simulink model "energy_trading"  (R2024b)
settings: Solver=VariableStepAuto  StartTime=0.0  StopTime=0.1  RelTol=1e-3
undefined symbols (not defined in the file): Acid, Lead
libraries: spsSeriesRLCBranchLib x12, spsPVArrayLib x3, spsDiodeLib x3, spsVoltageMeasurementLib x3, spsBatteryLib x2, spsMosfetLib x2, simulink x2, spsCurrentMeasurementLib x1, spsIGBTDiodeLib x1, spsPWMGenerator2LevelLib x1, spsUniversalBridgeLib x1, sps_lib x1
settings Model: Creator=ASUS  LastModifiedBy=ASUS

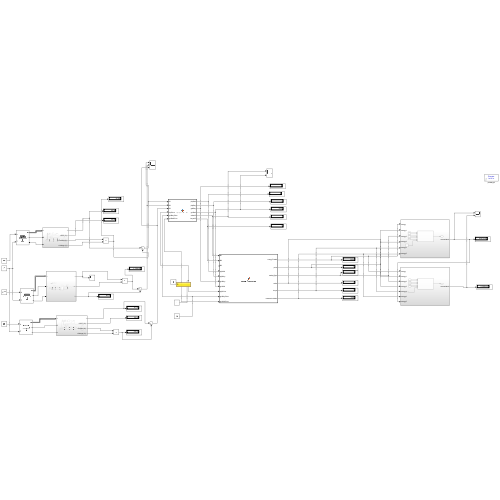
[thumbnail: Simulink's stored preview of the top-level diagram]
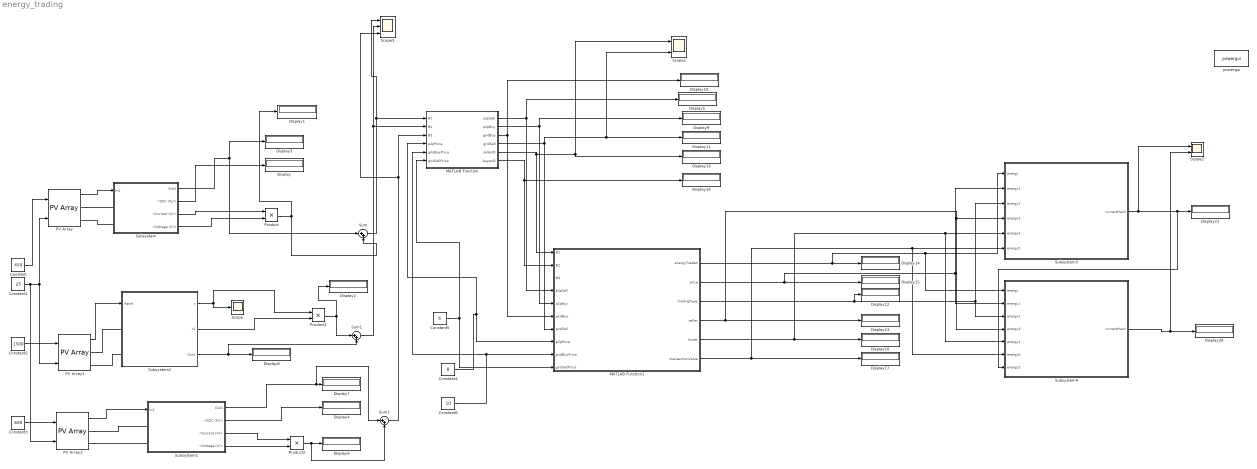
== system energy_trading ==
  Constant : Constant  Value=450
  Constant1 : Constant  Value=25
  Constant2 : Constant  Value=1500
  Constant3 : Constant  Value=600
  Constant4 : Constant  Value=8
  Constant5 : Constant  Value=6
  Constant6 : Constant  Value=10
  Display{,1..21} (22 alike) : Display
  MATLAB Function : MATLAB Function  TreatAsAtomicUnit=on
  MATLAB Function1 : MATLAB Function  TreatAsAtomicUnit=on
  PV Array : spsPVArrayLib/PV Array  Npar=1  Nser=1  PlotType=array @ 1000 W/m2 & specified temperatures  S_vec="[ 1000  500  100 ]"  Temp_C_vec="[ 45 25  ]"  ModuleName=User-defined  PlotWhenSelected=off  Pm=213.15  Ncell=60  Voc=36.3  Isc=7.84  Vm=29  Im=7.35  beta_Voc_pc=-0.36099  alpha_Isc_pc=0.102  beta_Voc=-0.13104  alpha_Isc=0.0079968  IL=7.8654  I0=2.9273e-10  nI=0.98119  Rsh=313.0553  Rs=0.39381  RobustModel=off  RobustCellTemperature=313.3991  BAL=on  Tc=1e-6  Tfilter=5e-5
  PV Array1 : spsPVArrayLib/PV Array  Npar=1  Nser=1  PlotType=array @ 1000 W/m2 & specified temperatures  S_vec="[ 1000  500  100 ]"  Temp_C_vec="[ 45 25  ]"  ModuleName=User-defined  PlotWhenSelected=off  Pm=213.15  Ncell=60  Voc=36.3  Isc=7.84  Vm=29  Im=7.35  beta_Voc_pc=-0.36099  alpha_Isc_pc=0.102  beta_Voc=-0.13104  alpha_Isc=0.0079968  IL=7.8654  I0=2.9273e-10  nI=0.98119  Rsh=313.0553  Rs=0.39381  RobustModel=off  RobustCellTemperature=313.3991  BAL=on  Tc=1e-6  Tfilter=5e-5
  PV Array2 : spsPVArrayLib/PV Array  Npar=1  Nser=1  PlotType=array @ 1000 W/m2 & specified temperatures  S_vec="[ 1000  500  100 ]"  Temp_C_vec="[ 45 25  ]"  ModuleName=User-defined  PlotWhenSelected=off  Pm=213.15  Ncell=60  Voc=36.3  Isc=7.84  Vm=29  Im=7.35  beta_Voc_pc=-0.36099  alpha_Isc_pc=0.102  beta_Voc=-0.13104  alpha_Isc=0.0079968  IL=7.8654  I0=2.9273e-10  nI=0.98119  Rsh=313.0553  Rs=0.39381  RobustModel=off  RobustCellTemperature=313.3991  BAL=on  Tc=1e-6  Tfilter=5e-5
  Product : Product
  Product1 : Product
  Product2 : Product
  Scope : Scope
  Scope1 : Scope  NumInputPorts=2
  Scope2 : Scope  NumInputPorts=2
  Scope3 : Scope  NumInputPorts=3
  Subsystem : Subsystem
  Subsystem1 : Subsystem
  Subsystem2 : Subsystem
  Subsystem3 : Subsystem
  Subsystem4 : Subsystem
  Sum : Sum  Inputs=|++
  Sum1 : Sum  Inputs=|++
  Sum2 : Sum  Inputs=|++
  powergui : sps_lib/powergui  Priority=1  SimulationMode=Discrete  SampleTime=1e-06  frequency=60  Iterations=50  frequencyindice=0  Pbase=100e6  ErrMax=1e-4  UnitsV=kV  UnitsW=MW  buscounter=0  FunctionMessages=off  echomessages=off  EnableUseOfTLC=off  CurrentSourceSwitches=off  DisableSnubberDevices=off  DisableRonSwitches=off  DisableVfSwitches=off  DisplayEquations=off  AutomaticDiscreteSolvers=off  SolverType=Tustin/Backward Euler (TBE)  Interpol=off  ExternalGateDelay=off  methode=off  Ts=100  x0status=blocks  SPID=on  SwTol=0  HookPort=off  NonlinearTolerance=1e-4  nMaxIteration=100  ContinueOnMaxIteration=off  RestoreLinks=warning  ResistiveCurrentMeasurement=off  Frange=[0:2:500]  Ylog=off  Xlog=on  ShowGrid=off  save=off  variable=ZData  structure=0  ZoomFFT=off  StartTime=0.0  cycles=1  DisplayStyle=1  fundamental=60  FreqAxis=off  MaxFrequency=1000  frequencyindicesteady=1  RmsSteady=1  display=off
  wires:
  Constant/1 -> PV Array/1
  Constant1/1 -> PV Array2/2, PV Array1/2, PV Array/2
  Constant3/1 -> PV Array2/1
  Constant2/1 -> PV Array1/1
  PV Array/1 -> Subsystem/1(In1)
  Subsystem/1(Out1) -> Display3/1, Sum/1
  Subsystem/2(<SOC (%)>) -> Display/1
  Subsystem/3(<Current (A)>) -> Product/1
  Subsystem/4(<Voltage (V)>) -> Product/2
  PV Array2/1 -> Subsystem1/1(In1)
  Subsystem1/1(Out1) -> Sum2/1, Display7/1
  Subsystem1/2(<SOC (%)>) -> Display4/1
  Subsystem2/1(v) -> Scope/1, Product1/1
  Product/1 -> Sum/2, Display1/1
  Subsystem2/2(c1) -> Product1/2
  Product1/1 -> Sum1/1, Display2/1
  PV Array1/1 -> Subsystem2/1(Inport)
  Subsystem2/3(Out1) -> Sum1/2, Display8/1
  Product2/1 -> Sum2/2, Display6/1
  Subsystem1/3(<Current (A)>) -> Product2/1
  Subsystem1/4(<Voltage (V)>) -> Product2/2
  MATLAB Function/1(p2pSell) -> Display5/1, MATLAB Function1/4(p2pSell)
  MATLAB Function/2(p2pBuy) -> Display9/1, MATLAB Function1/5(p2pBuy)
  MATLAB Function/3(gridBuy) -> Display10/1, MATLAB Function1/6(gridBuy)
  MATLAB Function/4(gridSell) -> Scope1/2, Display11/1, MATLAB Function1/7(gridSell)
  Constant5/1 -> MATLAB Function/6(gridSellPrice), MATLAB Function1/10(gridSellPrice)
  Constant6/1 -> MATLAB Function/5(gridBuyPrice), MATLAB Function1/9(gridBuyPrice)
  Constant4/1 -> MATLAB Function/4(p2pPrice), MATLAB Function1/8(p2pPrice)
  MATLAB Function1/3(tradingType) -> Display12/1, Subsystem4/3(energy2), Subsystem3/3(energy2)
  MATLAB Function1/4(seller) -> Subsystem4/4(energy3), Subsystem3/4(energy3), Display13/1
  MATLAB Function1/1(energyTraded) -> Subsystem4/1(energy), Subsystem3/1(energy), Display14/1
  MATLAB Function1/2(price) -> Subsystem4/2(energy1), Subsystem3/2(energy1), Display15/1
  MATLAB Function1/5(buyer) -> Subsystem4/5(energy4), Subsystem3/5(energy4), Display16/1
  MATLAB Function1/6(transactionValue) -> Subsystem4/6(energy6), Subsystem3/6(energy5), Display17/1
  MATLAB Function/5(sellerID) -> MATLAB Function1/1(B1), Display19/1, Scope1/1
  MATLAB Function/6(buyerID) -> MATLAB Function1/2(B2), Display18/1
  Subsystem3/1(currentHash) -> Scope2/1, Subsystem4/7(energy5), Display21/1
  Subsystem4/1(currentHash) -> Scope2/2, Display20/1
  Sum/1 -> Scope3/1, MATLAB Function/1(B1)
  Sum1/1 -> Scope3/2, MATLAB Function/2(B2)
  Sum2/1 -> Scope3/3, MATLAB Function/3(B3)
  connections:
  PV Array/RConn1 -- Subsystem/LConn1
  Subsystem/LConn2 -- PV Array/RConn2
  PV Array2/RConn1 -- Subsystem1/LConn1
  PV Array2/RConn2 -- Subsystem1/LConn2
  PV Array1/RConn1 -- Subsystem2/LConn1
  Subsystem2/LConn2 -- PV Array1/RConn2

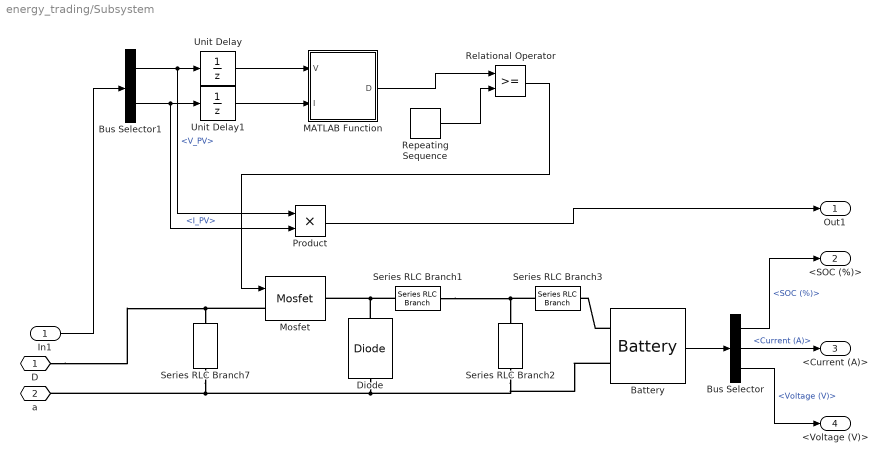
== system energy_trading/Subsystem ==
  In1 : Inport
  Battery : spsBatteryLib/Battery  BatType=Lead-Acid  NomV=12  NomQ=100  SOC=45  Batt_Tr=1  PresetModel=on  MaxQ=104.1667  MinV=9  FullV=13.0658  Dis_rate=20  R=0.0012  Normal_OP=31.0278  expZone="[12.2171     0.333333]"
  Bus Selector : BusSelector  OutputSignals=SOC (%),Current (A),Voltage (V)
  Bus Selector1 : BusSelector  OutputSignals=V_PV,I_PV
  Diode : spsDiodeLib/Diode  Ron=0.001  Lon=0  Vf=0.8  IC=0  UseSnubber=0  Rs=500  Cs=250e-9  Measurements=off
  MATLAB Function : MATLAB Function  TreatAsAtomicUnit=on
  Mosfet : spsMosfetLib/Mosfet  Ron=0.1  Lon=0  Rd=0.01  Vfd=0  IC=0  Rs=1e5  Cs=inf  Measurements=off
  Product : Product
  Relational Operator : RelationalOperator  OutDataTypeStr=boolean  RndMeth=Simplest  InputSameDT=off
  Repeating Sequence : simulink/Sources/Repeating Sequence  rep_seq_t=[0 0.0002]  rep_seq_y=[0 1]
  Series RLC Branch1 : spsSeriesRLCBranchLib/Series RLC Branch  LConnTagsString=__new0  RConnTagsString=__new0  BranchType=L  Resistance=0.0001  Inductance=0.783e-3  SetiL0=off  InitialCurrent=0  Capacitance=1000e-4  Setx0=off  InitialVoltage=0  Measurements=None
  Series RLC Branch2 : spsSeriesRLCBranchLib/Series RLC Branch  LConnTagsString=__new0  RConnTagsString=__new0  BranchType=C  Resistance=0.0001  Inductance=0.783e-3  SetiL0=off  InitialCurrent=0  Capacitance=364e-3  Setx0=off  InitialVoltage=0  Measurements=None
  Series RLC Branch3 : spsSeriesRLCBranchLib/Series RLC Branch  LConnTagsString=__new0  RConnTagsString=__new0  BranchType=R  Resistance=0.01  Inductance=0.783e-3  SetiL0=off  InitialCurrent=0  Capacitance=1000e-4  Setx0=off  InitialVoltage=0  Measurements=None
  Series RLC Branch7 : spsSeriesRLCBranchLib/Series RLC Branch  LConnTagsString=__new0  RConnTagsString=__new0  BranchType=RC  Resistance=0.0001  Inductance=1e-3  SetiL0=off  InitialCurrent=0  Capacitance=1000e-4  Setx0=off  InitialVoltage=0  Measurements=None
  Unit Delay : UnitDelay  SampleTime=1e-4  HasFrameUpgradeWarning=on
  Unit Delay1 : UnitDelay  SampleTime=1e-4  HasFrameUpgradeWarning=on
  D : PMIOPort  Side=Left
  a : PMIOPort  Port=2  Side=Left
  Out1 : Outport
  <SOC (%)> : Outport  Port=2
  <Current (A)> : Outport  Port=3
  <Voltage (V)> : Outport  Port=4
  wires:
  Battery/1 -> Bus Selector/1
  MATLAB Function/1(D) -> Relational Operator/1
  Bus Selector1/2 -> Product/2, Unit Delay1/1  "<I_PV>"
  Unit Delay1/1 -> MATLAB Function/2(I)
  Bus Selector1/1 -> Product/1, Unit Delay/1  "<V_PV>"
  Product/1 -> Out1/1
  Relational Operator/1 -> Mosfet/1
  Unit Delay/1 -> MATLAB Function/1(V)
  Repeating Sequence/1 -> Relational Operator/2
  Bus Selector/1 -> <SOC (%)>/1  "<SOC (%)>"
  In1/1 -> Bus Selector1/1
  Bus Selector/2 -> <Current (A)>/1  "<Current (A)>"
  Bus Selector/3 -> <Voltage (V)>/1  "<Voltage (V)>"
  connections:
  Series RLC Branch7/RConn1 -- a/RConn1 -- Battery/LConn2 -- Series RLC Branch2/LConn1 -- Diode/LConn1
  Series RLC Branch1/LConn1 -- Series RLC Branch2/RConn1 -- Series RLC Branch3/RConn1
  Diode/RConn1 -- Series RLC Branch1/RConn1 -- Mosfet/RConn1
  Battery/LConn1 -- Series RLC Branch3/LConn1
  Mosfet/LConn1 -- D/RConn1 -- Series RLC Branch7/LConn1

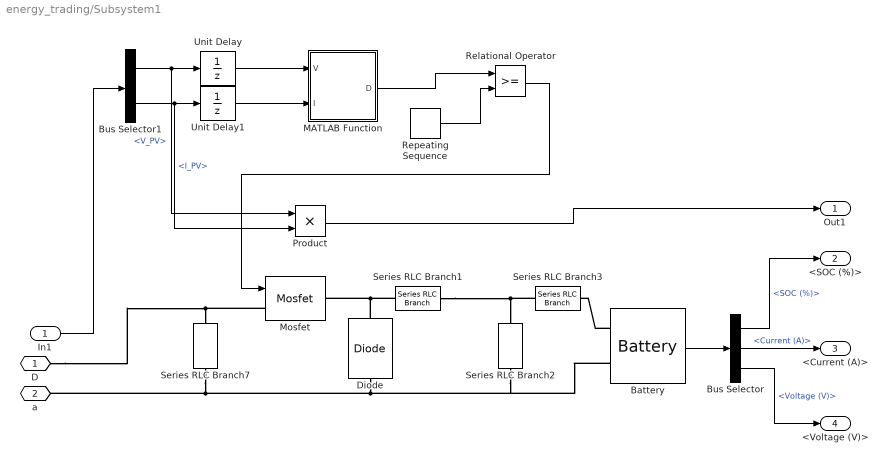
== system energy_trading/Subsystem1 ==
  In1 : Inport
  Battery : spsBatteryLib/Battery  BatType=Lead-Acid  NomV=12  NomQ=100  SOC=45  Batt_Tr=1  PresetModel=on  MaxQ=104.1667  MinV=9  FullV=13.0658  Dis_rate=20  R=0.0012  Normal_OP=31.0278  expZone="[12.2171     0.333333]"
  Bus Selector : BusSelector  OutputSignals=SOC (%),Current (A),Voltage (V)
  Bus Selector1 : BusSelector  OutputSignals=V_PV,I_PV
  Diode : spsDiodeLib/Diode  Ron=0.001  Lon=0  Vf=0.8  IC=0  UseSnubber=0  Rs=500  Cs=250e-9  Measurements=off
  MATLAB Function : MATLAB Function  TreatAsAtomicUnit=on
  Mosfet : spsMosfetLib/Mosfet  Ron=0.1  Lon=0  Rd=0.01  Vfd=0  IC=0  Rs=1e5  Cs=inf  Measurements=off
  Product : Product
  Relational Operator : RelationalOperator  OutDataTypeStr=boolean  RndMeth=Simplest  InputSameDT=off
  Repeating Sequence : simulink/Sources/Repeating Sequence  rep_seq_t=[0 0.0002]  rep_seq_y=[0 1]
  Series RLC Branch1 : spsSeriesRLCBranchLib/Series RLC Branch  LConnTagsString=__new0  RConnTagsString=__new0  BranchType=L  Resistance=0.0001  Inductance=0.783e-3  SetiL0=off  InitialCurrent=0  Capacitance=1000e-4  Setx0=off  InitialVoltage=0  Measurements=None
  Series RLC Branch2 : spsSeriesRLCBranchLib/Series RLC Branch  LConnTagsString=__new0  RConnTagsString=__new0  BranchType=C  Resistance=0.0001  Inductance=0.783e-3  SetiL0=off  InitialCurrent=0  Capacitance=364e-3  Setx0=off  InitialVoltage=0  Measurements=None
  Series RLC Branch3 : spsSeriesRLCBranchLib/Series RLC Branch  LConnTagsString=__new0  RConnTagsString=__new0  BranchType=R  Resistance=0.01  Inductance=0.783e-3  SetiL0=off  InitialCurrent=0  Capacitance=1000e-4  Setx0=off  InitialVoltage=0  Measurements=None
  Series RLC Branch7 : spsSeriesRLCBranchLib/Series RLC Branch  LConnTagsString=__new0  RConnTagsString=__new0  BranchType=RC  Resistance=0.0001  Inductance=1e-3  SetiL0=off  InitialCurrent=0  Capacitance=1000e-4  Setx0=off  InitialVoltage=0  Measurements=None
  Unit Delay : UnitDelay  SampleTime=1e-4  HasFrameUpgradeWarning=on
  Unit Delay1 : UnitDelay  SampleTime=1e-4  HasFrameUpgradeWarning=on
  D : PMIOPort  Side=Left
  a : PMIOPort  Port=2  Side=Left
  Out1 : Outport
  <SOC (%)> : Outport  Port=2
  <Current (A)> : Outport  Port=3
  <Voltage (V)> : Outport  Port=4
  wires:
  Battery/1 -> Bus Selector/1
  MATLAB Function/1(D) -> Relational Operator/1
  Bus Selector1/2 -> Product/2, Unit Delay1/1  "<I_PV>"
  Unit Delay1/1 -> MATLAB Function/2(I)
  Bus Selector1/1 -> Product/1, Unit Delay/1  "<V_PV>"
  Product/1 -> Out1/1
  Relational Operator/1 -> Mosfet/1
  Unit Delay/1 -> MATLAB Function/1(V)
  Repeating Sequence/1 -> Relational Operator/2
  Bus Selector/1 -> <SOC (%)>/1  "<SOC (%)>"
  In1/1 -> Bus Selector1/1
  Bus Selector/2 -> <Current (A)>/1  "<Current (A)>"
  Bus Selector/3 -> <Voltage (V)>/1  "<Voltage (V)>"
  connections:
  Series RLC Branch7/RConn1 -- Series RLC Branch2/LConn1 -- Battery/LConn2 -- Diode/LConn1 -- a/RConn1
  Series RLC Branch1/LConn1 -- Series RLC Branch3/RConn1 -- Series RLC Branch2/RConn1
  Diode/RConn1 -- Mosfet/RConn1 -- Series RLC Branch1/RConn1
  Battery/LConn1 -- Series RLC Branch3/LConn1
  Mosfet/LConn1 -- D/RConn1 -- Series RLC Branch7/LConn1

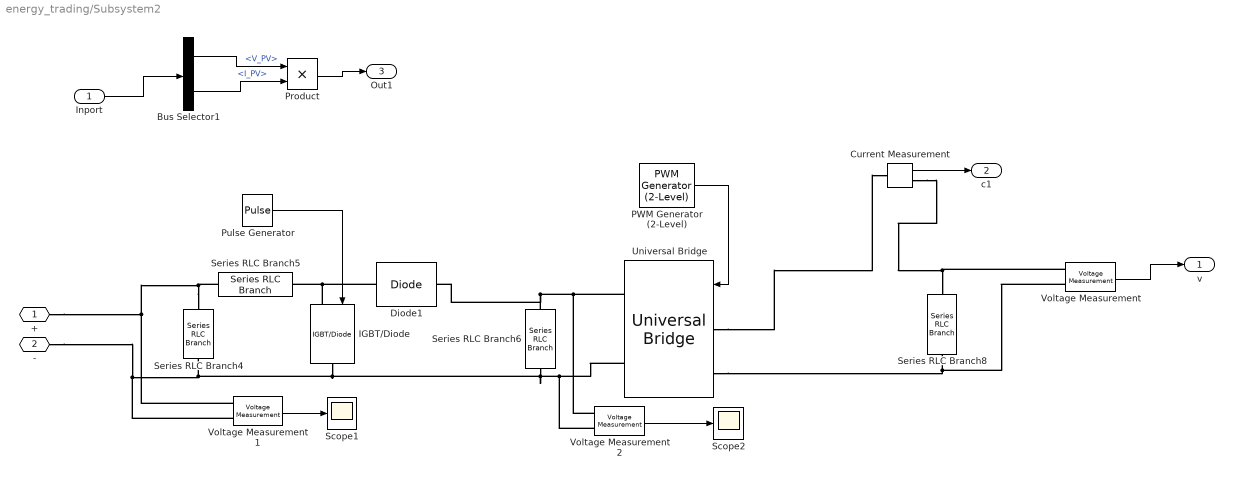
== system energy_trading/Subsystem2 ==
  Inport : Inport
  Bus Selector1 : BusSelector  OutputSignals=V_PV,I_PV
  Current Measurement : spsCurrentMeasurementLib/Current Measurement  PhasorSimulation=off  OutputType=Complex  PSBequivalent=0
  Diode1 : spsDiodeLib/Diode  Ron=0.001  Lon=0  Vf=0.8  IC=0  UseSnubber=0  Rs=500  Cs=250e-9  Measurements=off
  IGBT/Diode : spsIGBTDiodeLib/IGBT//Diode  Ron=1e-3  Rs=1e5  Cs=inf  Measurements=off
  PWM Generator (2-Level) : spsPWMGenerator2LevelLib/PWM Generator (2-Level)  ModulatorType=Single-phase full-bridge (4 pulses)  ModulatorMode=Unsynchronized  Fc=27*60  Pc=90  nF=27  MinMax="[ -1  1 ]"  SamplingTechnique=Natural  ModulatingSignals=on  m=0.8  Freq=60  Phase=0  Ts=0  ShowCarrierOutport=off
  Product : Product
  Pulse Generator : DiscretePulseGenerator  PulseType=Time based  Period=1/1500  PulseWidth=50
  Scope1 : Scope
  Scope2 : Scope
  Series RLC Branch4 : spsSeriesRLCBranchLib/Series RLC Branch  LConnTagsString=__new0  RConnTagsString=__new0  BranchType=C  Resistance=0.0001  Inductance=1e-3  SetiL0=off  InitialCurrent=0  Capacitance=0.006  Setx0=off  InitialVoltage=0  Measurements=None
  Series RLC Branch5 : spsSeriesRLCBranchLib/Series RLC Branch  LConnTagsString=__new0  RConnTagsString=__new0  BranchType=L  Resistance=0.0001  Inductance=0.02  SetiL0=off  InitialCurrent=0  Capacitance=0.006  Setx0=off  InitialVoltage=0  Measurements=None
  Series RLC Branch6 : spsSeriesRLCBranchLib/Series RLC Branch  LConnTagsString=__new0  RConnTagsString=__new0  BranchType=C  Resistance=0.0001  Inductance=1e-3  SetiL0=off  InitialCurrent=0  Capacitance=0.006  Setx0=off  InitialVoltage=0  Measurements=None
  Series RLC Branch8 : spsSeriesRLCBranchLib/Series RLC Branch  LConnTagsString=__new0  RConnTagsString=__new0  BranchType=L  Resistance=0.0001  Inductance=50  SetiL0=off  InitialCurrent=0  Capacitance=0.006  Setx0=off  InitialVoltage=0  Measurements=None
  Universal Bridge : spsUniversalBridgeLib/Universal Bridge  Arms=2  SnubberResistance=1e5  SnubberCapacitance=inf  Device=IGBT / Diodes  Ron=1e-3  Lon=0  ForwardVoltages="[  0  0  ]"  ForwardVoltage=0  GTOparameters=[ 10e-6 , 20e-6 ]  IGBTparameters=[ 1e-6 , 2e-6 ]  Measurements=None  Measurements_2=None  converterType=Rectifier
  Voltage Measurement : spsVoltageMeasurementLib/Voltage Measurement  PhasorSimulation=off  OutputType=Complex  PSBequivalent=0
  Voltage Measurement1 : spsVoltageMeasurementLib/Voltage Measurement  PhasorSimulation=off  OutputType=Complex  PSBequivalent=0
  Voltage Measurement2 : spsVoltageMeasurementLib/Voltage Measurement  PhasorSimulation=off  OutputType=Complex  PSBequivalent=0
  + : PMIOPort  Side=Left
  - : PMIOPort  Port=2  Side=Left
  v : Outport
  c1 : Outport  Port=2
  Out1 : Outport  Port=3
  wires:
  PWM Generator (2-Level)/1 -> Universal Bridge/1
  Pulse Generator/1 -> IGBT/Diode/1
  Voltage Measurement1/1 -> Scope1/1
  Voltage Measurement2/1 -> Scope2/1
  Voltage Measurement/1 -> v/1
  Current Measurement/1 -> c1/1
  Inport/1 -> Bus Selector1/1
  Bus Selector1/1 -> Product/1  "<V_PV>"
  Bus Selector1/2 -> Product/2  "<I_PV>"
  Product/1 -> Out1/1
  connections:
  Voltage Measurement/LConn1 -- Current Measurement/RConn1 -- Series RLC Branch8/LConn1
  Series RLC Branch6/LConn1 -- Universal Bridge/RConn1 -- Voltage Measurement2/LConn1 -- Diode1/RConn1
  Series RLC Branch4/LConn1 -- +/RConn1 -- Voltage Measurement1/LConn1 -- Series RLC Branch5/RConn1
  Universal Bridge/LConn2 -- Voltage Measurement/LConn2 -- Series RLC Branch8/RConn1
  Series RLC Branch4/RConn1 -- Voltage Measurement2/LConn2 -- Universal Bridge/RConn2 -- Series RLC Branch6/RConn1 -- IGBT/Diode/RConn1 -- -/RConn1 -- Voltage Measurement1/LConn2
  Diode1/LConn1 -- Series RLC Branch5/LConn1 -- IGBT/Diode/LConn1
  Universal Bridge/LConn1 -- Current Measurement/LConn1

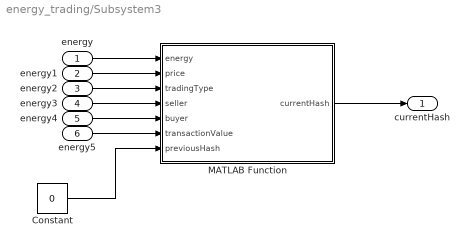
== system energy_trading/Subsystem3 ==
  energy : Inport
  energy1 : Inport  Port=2
  energy2 : Inport  Port=3
  energy3 : Inport  Port=4
  energy4 : Inport  Port=5
  energy5 : Inport  Port=6
  Constant : Constant  Value=0
  MATLAB Function : MATLAB Function  TreatAsAtomicUnit=on
  currentHash : Outport
  wires:
  Constant/1 -> MATLAB Function/7(previousHash)
  energy/1 -> MATLAB Function/1(energy)
  energy1/1 -> MATLAB Function/2(price)
  energy2/1 -> MATLAB Function/3(tradingType)
  energy3/1 -> MATLAB Function/4(seller)
  energy4/1 -> MATLAB Function/5(buyer)
  energy5/1 -> MATLAB Function/6(transactionValue)
  MATLAB Function/1(currentHash) -> currentHash/1

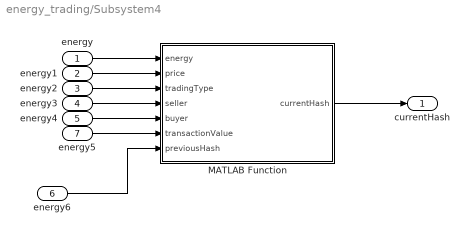
== system energy_trading/Subsystem4 ==
  energy : Inport
  energy1 : Inport  Port=2
  energy2 : Inport  Port=3
  energy3 : Inport  Port=4
  energy4 : Inport  Port=5
  energy6 : Inport  Port=6
  energy5 : Inport  Port=7
  MATLAB Function : MATLAB Function  TreatAsAtomicUnit=on
  currentHash : Outport
  wires:
  energy/1 -> MATLAB Function/1(energy)
  energy1/1 -> MATLAB Function/2(price)
  energy2/1 -> MATLAB Function/3(tradingType)
  energy3/1 -> MATLAB Function/4(seller)
  energy4/1 -> MATLAB Function/5(buyer)
  energy5/1 -> MATLAB Function/6(transactionValue)
  MATLAB Function/1(currentHash) -> currentHash/1
  energy6/1 -> MATLAB Function/7(previousHash)

== matlab function energy_trading/Subsystem1/MATLAB Function ==
  data: V input; D output; I input
function D=DutyRation(V,I)
Dmax=0.95;
Dmin=0;
Dinit=0.95;
deltaD=0.0001;
persistent Vold Pold Dold;

dataType='double';

if isempty(Vold)
    Vold=0;
    Pold=0;
    Dold=Dinit;
end
P=V*I;
dV=V-Vold;
dP=P-Pold;
if dP~=0
    if dP<0
        if dV<0
            D=Dold-deltaD;
        else
            D=Dold+deltaD;
        end
    else
        if dV<0
            D=Dold+deltaD;
        else
            D=Dold-deltaD;
        end
    end
else D=Dold;
end
if D>=Dmax||D<=Dmin
    D=Dold;
end
Dold=D;
Vold=V;
Pold=P;

== matlab function energy_trading/Subsystem/MATLAB Function ==
  data: V input; D output; I input
function D=DutyRation(V,I)
Dmax=0.95;
Dmin=0;
Dinit=0.95;
deltaD=0.0001;
persistent Vold Pold Dold;

dataType='double';

if isempty(Vold)
    Vold=0;
    Pold=0;
    Dold=Dinit;
end
P=V*I;
dV=V-Vold;
dP=P-Pold;
if dP~=0
    if dP<0
        if dV<0
            D=Dold-deltaD;
        else
            D=Dold+deltaD;
        end
    else
        if dV<0
            D=Dold+deltaD;
        else
            D=Dold-deltaD;
        end
    end
else D=Dold;
end
if D>=Dmax||D<=Dmin
    D=Dold;
end
Dold=D;
Vold=V;
Pold=P;

== matlab function energy_trading/MATLAB Function ==
  data: p2pSell output; p2pBuy output; gridBuy output; gridSell output; B1 input; B2 input; B3 input; p2pPrice input; gridBuyPrice input; gridSellPrice input; sellerID output; buyerID output
function [p2pSell,p2pBuy,gridBuy,gridSell,sellerID,buyerID] = adaptiveTrading(B1,B2,B3,p2pPrice,gridBuyPrice,gridSellPrice)

% Participant balances
% Positive = surplus
% Negative = deficit

B = [B1 B2 B3];

% Calculate total surplus and deficit
surplus = max(B1,0) + max(B2,0) + max(B3,0);
deficit = max(-B1,0) + max(-B2,0) + max(-B3,0);

% Initialize outputs
p2pSell = 0;
p2pBuy  = 0;
gridBuy  = 0;
gridSell = 0;

sellerID = 0;
buyerID  = 0;

% Check whether P2P trading is economically beneficial
if (p2pPrice > gridSellPrice) && (p2pPrice < gridBuyPrice)

    % Amount that can be traded through P2P
    p2pPower = min(surplus,deficit);

    p2pSell = p2pPower;
    p2pBuy  = p2pPower;

    % Remaining energy goes to/from grid
    gridBuy  = deficit - p2pPower;
    gridSell = surplus - p2pPower;

    % Find seller
    for i = 1:3
        if B(i) > 0
            sellerID = i;
            break;
        end
    end

    % Find buyer
    for i = 1:3
        if B(i) < 0
            buyerID = i;
            break;
        end
    end

else

    % P2P is not economically beneficial
    gridBuy  = deficit;
    gridSell = surplus;

end

== matlab function energy_trading/MATLAB Function1 ==
  data: B1 input; B2 input; B3 input; p2pSell input; energyTraded output; p2pBuy input; gridBuy input; gridSell input; p2pPrice input; gridBuyPrice input; gridSellPrice input; price output; tradingType output; seller output; buyer output; transactionValue output
function [energyTraded, price, tradingType, seller, buyer, transactionValue] = ...
    energyTransaction(B1,B2,B3,p2pSell,p2pBuy,gridBuy,gridSell,...
                      p2pPrice,gridBuyPrice,gridSellPrice)

% Store participant balances
B = [B1 B2 B3];

% Initial values
energyTraded = 0;
price = 0;
tradingType = 0;
seller = 0;
buyer = 0;
transactionValue = 0;

%% P2P Transaction
if p2pSell > 0 && p2pBuy > 0

    energyTraded = min(p2pSell,p2pBuy);
    price = p2pPrice;
    tradingType = 1;       % 1 = P2P

    % Find first surplus participant
    for i = 1:3
        if B(i) > 0
            seller = i;
            break;
        end
    end

    % Find first deficit participant
    for j = 1:3
        if B(j) < 0
            buyer = j;
            break;
        end
    end

    transactionValue = energyTraded * price;

%% Grid Buy
elseif gridBuy > 0

    energyTraded = gridBuy;
    price = gridBuyPrice;
    tradingType = 2;       % 2 = Grid Buy

    seller = 0;            % Grid
    buyer = 0;             % Grid transaction

    transactionValue = energyTraded * price;

%% Grid Sell
elseif gridSell > 0

    energyTraded = gridSell;
    price = gridSellPrice;
    tradingType = 3;       % 3 = Grid Sell

    seller = 0;            % Participant-to-grid
    buyer = 0;             % Grid

    transactionValue = energyTraded * price;

end

== matlab function energy_trading/Subsystem3/MATLAB Function ==
  data: energy input; currentHash output; price input; tradingType input; seller input; buyer input; transactionValue input; previousHash input

function currentHash = generateHash(energy,price,tradingType, ...
    seller,buyer,transactionValue,previousHash)

% Simple numeric hash for Simulink demonstration
% Inputs must match energyTransaction outputs

data = [energy; price; tradingType; seller; buyer; ...
        transactionValue; previousHash];

% Weighted calculation to distinguish input positions
weights = [11; 17; 23; 31; 41; 53; 67];

weightedData = sum(data .* weights);

currentHash = mod(weightedData * 1009 + 12345, 1000000);

end

== matlab function energy_trading/Subsystem4/MATLAB Function ==
  data: energy input; currentHash output; price input; tradingType input; seller input; buyer input; transactionValue input; previousHash input

function currentHash = generateHash(energy,price,tradingType, ...
    seller,buyer,transactionValue,previousHash)

% Simple numeric hash for Simulink demonstration
% Inputs must match energyTransaction outputs

data = [energy; price; tradingType; seller; buyer; ...
        transactionValue; previousHash];

% Weighted calculation to distinguish input positions
weights = [11; 17; 23; 31; 41; 53; 67];

weightedData = sum(data .* weights);

currentHash = mod(weightedData * 1009 + 12345, 1000000);

end
